simulink model "scheme_L2"  (R2026b)
settings: Solver=ode4  StopTime=10  FixedStep=1e-3
settings Model: Creator=Ernest  LastModifiedBy=Ernest

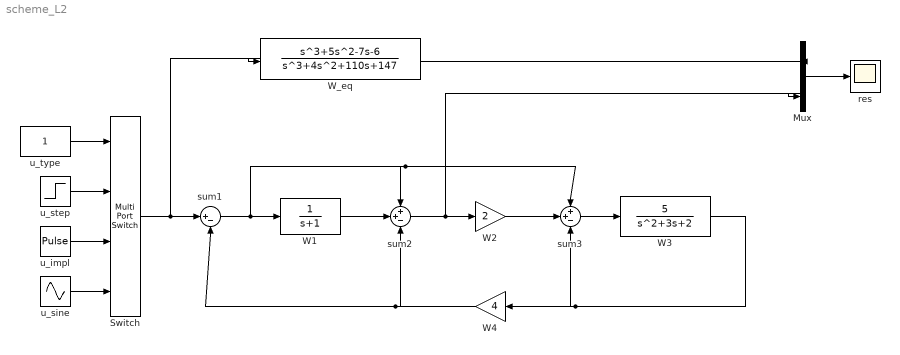
== system scheme_L2 ==
  u_type : Constant  Value=1
  u_step : Step  Time=0  SampleTime=0
  u_impl : DiscretePulseGenerator  PulseType=Time based  Amplitude=10  Period=20  PulseWidth=0.5  PhaseDelay=0
  u_sine : Sin  Frequency=2  SampleTime=0
  Switch : MultiPortSwitch
  sum1 : Sum  Inputs=|+-
  W1 : TransferFcn  Denominator=[1 1]
  sum2 : Sum  Inputs=++-
  W2 : Gain  Gain=2
  sum3 : Sum  Inputs=++-
  W3 : TransferFcn  Numerator=[5]  Denominator=[1 3 2]
  W4 : Gain  Gain=4
  W_eq : TransferFcn  Numerator=[1 5 -7 -6]  Denominator=[1 4 110 147]
  Mux : Mux  Inputs=2
  res : Scope
  wires:
  u_type/1 -> Switch/1
  u_step/1 -> Switch/2
  u_impl/1 -> Switch/3
  u_sine/1 -> Switch/4
  Switch/1 -> sum1/1, W_eq/1
  sum1/1 -> W1/1, sum2/1, sum3/1
  W1/1 -> sum2/2
  sum2/1 -> W2/1, Mux/2
  W2/1 -> sum3/2
  sum3/1 -> W3/1
  W3/1 -> sum3/3, W4/1
  W4/1 -> sum2/3, sum1/2
  W_eq/1 -> Mux/1
  Mux/1 -> res/1
